simulink model "test"  (R2018b)
settings: Solver=VariableStepAuto  StartTime=0.0  StopTime=inf  RelTol=1e-3
undefined symbols (not defined in the file or in its folder): DD, NN, PP, RR
settings Model: Creator=19810  LastModifiedBy=19810

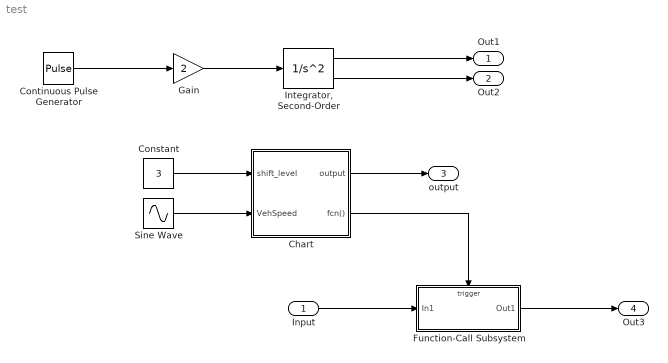
== system test ==
  Input : Inport
  Chart : Stateflow chart  TreatAsAtomicUnit=on
  Constant : Constant  Value=3
  Continuous Pulse Generator : DiscretePulseGenerator  PulseType=Time based  Period=1  PulseWidth=50
  Function-Call Subsystem : Subsystem  TreatAsAtomicUnit=on
  Gain : Gain  Gain=2
  "Integrator, Second-Order" : SecondOrderIntegrator
  Sine Wave : Sin  Amplitude=80  SampleTime=0
  Out1 : Outport
  Out2 : Outport  Port=2
  output : Outport  Port=3
  Out3 : Outport  Port=4
  wires:
  "Integrator, Second-Order"/1 -> Out1/1
  "Integrator, Second-Order"/2 -> Out2/1
  Continuous Pulse Generator/1 -> Gain/1
  Gain/1 -> "Integrator, Second-Order"/1
  Sine Wave/1 -> Chart/2(VehSpeed)
  Chart/1(output) -> output/1
  Constant/1 -> Chart/1(shift_level)
  Input/1 -> Function-Call Subsystem/1(In1)
  Function-Call Subsystem/1(Out1) -> Out3/1
  Chart/2(fcn()) -> Function-Call Subsystem/Trigger

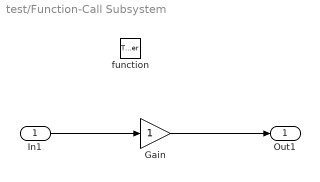
== system test/Function-Call Subsystem ==
  In1 : Inport
  function : TriggerPort  TriggerType=function-call  VariantControl=Variant
  Gain : Gain
  Out1 : Outport
  wires:
  In1/1 -> Gain/1
  Gain/1 -> Out1/1

== stateflow chart test/Chart ==
  state R
    en:
    fcn
    du:
    fcn
  state D
    state D1
      en:
      output=10;
    state D2
      en:
      output=20;
    state D3
      en:
      output=30;
    state D4
      en:
      output=40;
    (default) -> D1
    D3 -> D4 [order 2] : [VehSpeed>70]
    D2 -> D3 [order 2] : [VehSpeed>50]
    D1 -> D2 : [VehSpeed>30]
    D4 -> D3 : [VehSpeed<65]
    D2 -> D1 [order 1] : [VehSpeed<25]
    D3 -> D2 [order 1] : [VehSpeed<45]
  state P
  state N
  (default) -> P
  R -> N [order 1] : [shift_level==NN]
  N -> D [order 1] : [shift_level==DD]
  P -> R : [shift_level==RR]
  D -> N : [shift_level==NN]
  N -> R [order 2] : [shift_level==RR]
  R -> P [order 2] : [shift_level==PP]
  data: shift_level input; output output; VehSpeed input; PP parameter; RR parameter; NN parameter; DD parameter
  events: fcn output FUNCTION_CALL_EVENT
